simulink model "exp6"  (R2026b)
settings: Solver=VariableStepAuto  StopTime=200

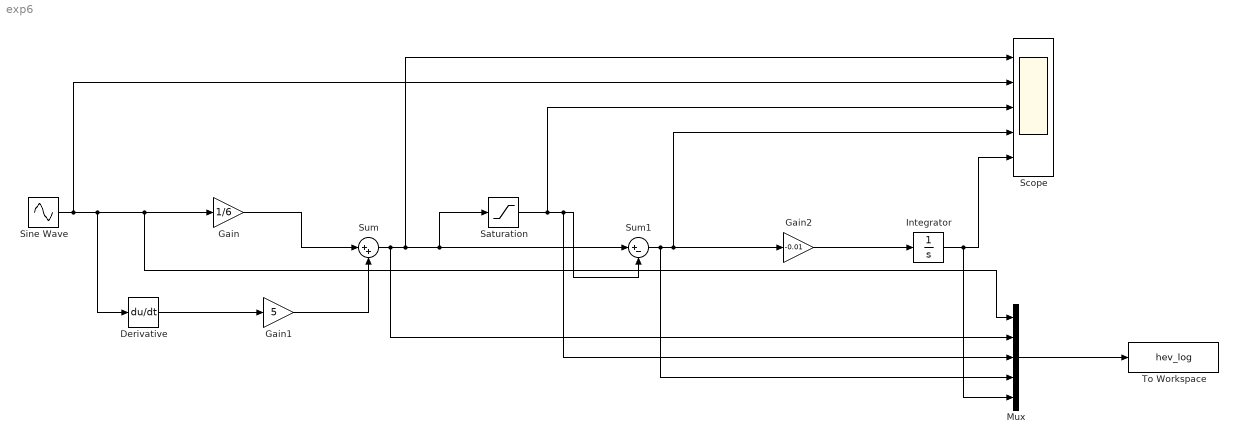
== system exp6 ==
  Derivative : Derivative
  Gain : Gain  Gain=1/6
  Gain1 : Gain  Gain=5
  Gain2 : Gain  Gain=-0.01
  Integrator : Integrator  InitialCondition=60
  Mux : Mux  Inputs=5
  Saturation : Saturate  UpperLimit=15  LowerLimit=0
  Scope : Scope  NumInputPorts=5
      settings: ActiveDisplayYMinimum=-237.71475351119091  ActiveDisplayYMaximum=201.54009984134427
  Sine Wave : Sin  Amplitude=40  Bias=50  Frequency=0.05  Phase=-pi/2  SampleTime=0
  Sum : Sum  Inputs=|++
  Sum1 : Sum  Inputs=|+-
  To Workspace : ToWorkspace  VariableName=hev_log  SaveFormat=Timeseries  SampleTime=-1
  wires:
  Sine Wave/1 -> Scope/2, Derivative/1, Mux/1, Gain/1
  Gain/1 -> Sum/1
  Gain1/1 -> Sum/2
  Sum/1 -> Mux/2, Scope/1, Saturation/1, Sum1/1
  Derivative/1 -> Gain1/1
  Saturation/1 -> Scope/3, Mux/3, Sum1/2
  Sum1/1 -> Mux/4, Scope/4, Gain2/1
  Gain2/1 -> Integrator/1
  Integrator/1 -> Mux/5, Scope/5
  Mux/1 -> To Workspace/1
